simulink model "CLLCTestHarnessPlant"  (R2026a)
settings: Solver=ode23t  StopTime=5e-3  FixedStep=1e-4  MaxStep=1e-6  AbsTol=1e-3
PreLoadFcn:
  | CLLCConverterDefaultInputParameters;
undefined symbols (not defined in the file or in its folder): CLLCCompensator, CLLCController, CLLCDesign, DiscIntNeverNeededParam
libraries: fl_lib x46, nesl_utility x45, ee_lib x35
(part 2 of 4)

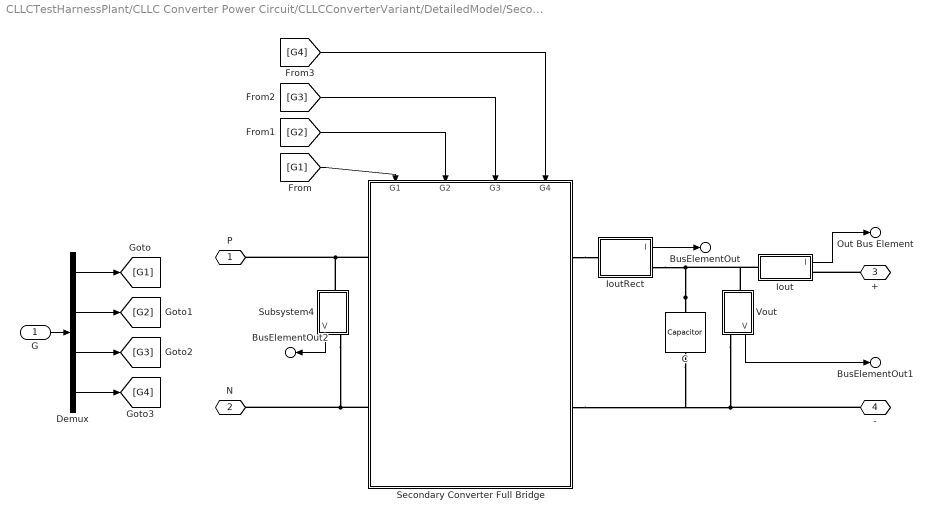
== system CLLCTestHarnessPlant/CLLC Converter Power Circuit/CLLCConverterVariant/DetailedModel/Secondary Converter ==
  G : Inport
  C : fl_lib/Electrical/Electrical Elements/Capacitor  c=Co F  r=Rco Ohm  g=0 1/Ohm  i_specify=off  i_priority=None  i=0 A  i_nominal_specify=off  i_nominal_value=1  i_nominal_unit=A  v_specify=off  v_priority=None  v=450 V  v_nominal_specify=off  v_nominal_value=1  v_nominal_unit=V  vc_specify=on  vc_priority=High  vc=Vco V  vc_nominal_specify=off  vc_nominal_value=1  vc_nominal_unit=V
  Demux : Demux
  Iout : Subsystem
      mask Display: disp("I")
  IoutRect : Subsystem
      mask Display: disp("I")
  Secondary Converter Full Bridge : Subsystem  Variant=on  VariantControlMode=label  LabelModeActiveChoice=IdealSwitch
      settings: PortSchema="{\"entries\":[{\"content\":{\"sides\":[{\"content\":{\"connectorIds\":[\"LConn1\",\"LConn2\"]},\"type\":\"ConnectorPlacement.EquallySpacedRectSide\",\"uuid\":\"27c41940-d662-4779-afdd-48b642f77411\"},{\"content\":{\"connectorIds\":[\"RConn1\",\"RConn2\"],\"side\":\"RIGHT\"},\"type\":\"ConnectorPlacement.EquallySpacedRectSide\",\"uuid\":\"b0072b01-add1-4b0f-b94e-e1b6c9886b0e\"},{\"content\":{\"connectorIds\":[\"In1\",\"In2\",\"In3\",\"In4\"],\"side\":\"TOP\"},\"type\":\"ConnectorPlacement.EquallySpacedRectSide\",\"uuid\":\"c43bed80-422d-49db-9596-8b38d5c3e411\"},{\"content\":{\"side\":\"BOTTOM\"},\"type\":\"ConnectorPlacement.EquallySpacedRectSide\",\"uuid\":\"01f06046-f57e-45b0-bca5-368a5a543f97\"}]},\"type\":\"ConnectorPlacement.EquallySpacedConnector\",\"uuid\":\"2fcb5370-6bd7-4702-bf87-ebedbb7e376c\"}],\"packageUris\":[\"http://schema.mathworks.com/mf0/Connector/R2020b\"],\"version\":\"1.0\"}"
  Subsystem4 : Subsystem
      settings: PortSchema="{\"entries\":[{\"content\":{\"sides\":[{\"content\":{\"connectorIds\":[\"LConn1\"]},\"type\":\"ConnectorPlacement.EquallySpacedRectSide\",\"uuid\":\"e749c2ff-fd60-426f-a769-b61a7dfe80d2\"},{\"content\":{\"connectorIds\":[\"RConn1\",\"Out1\"],\"side\":\"RIGHT\"},\"type\":\"ConnectorPlacement.EquallySpacedRectSide\",\"uuid\":\"f3bb02bd-f8d2-4326-b68c-6f969fa4ac22\"},{\"content\":{\"side\":\"TOP\"},\"type\":\"ConnectorPlacement.EquallySpacedRectSide\",\"uuid\":\"9ab7a0d1-20d8-49e4-8eb3-54d34434204c\"}]},\"type\":\"ConnectorPlacement.EquallySpacedConnector\",\"uuid\":\"19e2a6d5-13f4-47de-bb59-b826817cba83\"}],\"packageUris\":[\"http://schema.mathworks.com/mf0/Connector/R2020b\"],\"version\":\"1.0\"}"
      mask Display: disp("V")
  Vout : Subsystem
      settings: PortSchema="{\"entries\":[{\"content\":{\"sides\":[{\"content\":{\"connectorIds\":[\"LConn1\"]},\"type\":\"ConnectorPlacement.EquallySpacedRectSide\",\"uuid\":\"e749c2ff-fd60-426f-a769-b61a7dfe80d2\"},{\"content\":{\"connectorIds\":[\"RConn1\",\"Out1\"],\"side\":\"RIGHT\"},\"type\":\"ConnectorPlacement.EquallySpacedRectSide\",\"uuid\":\"f3bb02bd-f8d2-4326-b68c-6f969fa4ac22\"},{\"content\":{\"side\":\"TOP\"},\"type\":\"ConnectorPlacement.EquallySpacedRectSide\",\"uuid\":\"9ab7a0d1-20d8-49e4-8eb3-54d34434204c\"}]},\"type\":\"ConnectorPlacement.EquallySpacedConnector\",\"uuid\":\"19e2a6d5-13f4-47de-bb59-b826817cba83\"}],\"packageUris\":[\"http://schema.mathworks.com/mf0/Connector/R2020b\"],\"version\":\"1.0\"}"
      mask Display: disp("V")
  P : PMIOPort  Side=Left
  N : PMIOPort  Port=2  Side=Left
  + : PMIOPort  Port=3  Side=Right
  - : PMIOPort  Port=4  Side=Right
  Out Bus Element : Outport  PortName=meas  Element=Iout [A]
  BusElementOut : Outport  PortName=meas  Element=IL [A]
  BusElementOut1 : Outport  PortName=meas  Element=Vout [V]
  BusElementOut2 : Outport  PortName=meas  Element=Vac [V]
  wires:
  [G4] -> Secondary Converter Full Bridge/4(G4)
  [G1] -> Secondary Converter Full Bridge/1(G1)
  [G3] -> Secondary Converter Full Bridge/3(G3)
  [G2] -> Secondary Converter Full Bridge/2(G2)
  Demux/3 -> [G3]
  Demux/4 -> [G4]
  G/1 -> Demux/1
  Demux/1 -> [G1]
  Demux/2 -> [G2]
  Subsystem4/1(V) -> BusElementOut2/1
  Vout/1(V) -> BusElementOut1/1
  IoutRect/1(I) -> BusElementOut/1
  Iout/1(I) -> Out Bus Element/1
  connections:
  +/RConn1 -- Iout/RConn1
  C/LConn1 -- Vout/LConn1 -- Iout/LConn1 -- IoutRect/RConn1
  -/RConn1 -- Secondary Converter Full Bridge/RConn2 -- C/RConn1 -- Vout/RConn1
  Subsystem4/LConn1 -- Secondary Converter Full Bridge/LConn1 -- P/RConn1
  Subsystem4/RConn1 -- Secondary Converter Full Bridge/LConn2 -- N/RConn1
  Secondary Converter Full Bridge/RConn1 -- IoutRect/LConn1

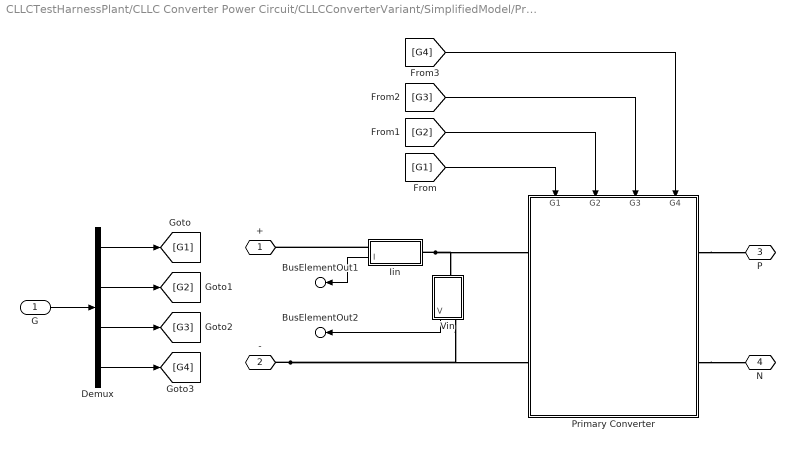
== system CLLCTestHarnessPlant/CLLC Converter Power Circuit/CLLCConverterVariant/SimplifiedModel/Primary Converter ==
  G : Inport
  Demux : Demux
  Iin : Subsystem
      settings: PortSchema="{\"entries\":[{\"content\":{\"sides\":[{\"content\":{\"connectorIds\":[\"LConn1\",\"Out1\"]},\"type\":\"ConnectorPlacement.EquallySpacedRectSide\",\"uuid\":\"e749c2ff-fd60-426f-a769-b61a7dfe80d2\"},{\"content\":{\"connectorIds\":[\"RConn1\"],\"side\":\"RIGHT\"},\"type\":\"ConnectorPlacement.EquallySpacedRectSide\",\"uuid\":\"f3bb02bd-f8d2-4326-b68c-6f969fa4ac22\"},{\"content\":{\"side\":\"TOP\"},\"type\":\"ConnectorPlacement.EquallySpacedRectSide\",\"uuid\":\"9ab7a0d1-20d8-49e4-8eb3-54d34434204c\"}]},\"type\":\"ConnectorPlacement.EquallySpacedConnector\",\"uuid\":\"19e2a6d5-13f4-47de-bb59-b826817cba83\"}],\"packageUris\":[\"http://schema.mathworks.com/mf0/Connector/R2020b\"],\"version\":\"1.0\"}"
      mask Display: disp("I")
  Primary Converter : Subsystem  VariantControl=IdealSwitch
      settings: PortSchema="{\"entries\":[{\"content\":{\"sides\":[{\"content\":{\"connectorIds\":[\"LConn1\",\"LConn2\"]},\"type\":\"ConnectorPlacement.EquallySpacedRectSide\",\"uuid\":\"27c41940-d662-4779-afdd-48b642f77411\"},{\"content\":{\"connectorIds\":[\"RConn1\",\"RConn2\"],\"side\":\"RIGHT\"},\"type\":\"ConnectorPlacement.EquallySpacedRectSide\",\"uuid\":\"b0072b01-add1-4b0f-b94e-e1b6c9886b0e\"},{\"content\":{\"connectorIds\":[\"In1\",\"In2\",\"In3\",\"In4\"],\"side\":\"TOP\"},\"type\":\"ConnectorPlacement.EquallySpacedRectSide\",\"uuid\":\"c43bed80-422d-49db-9596-8b38d5c3e411\"},{\"content\":{\"side\":\"BOTTOM\"},\"type\":\"ConnectorPlacement.EquallySpacedRectSide\",\"uuid\":\"01f06046-f57e-45b0-bca5-368a5a543f97\"}]},\"type\":\"ConnectorPlacement.EquallySpacedConnector\",\"uuid\":\"2fcb5370-6bd7-4702-bf87-ebedbb7e376c\"}],\"packageUris\":[\"http://schema.mathworks.com/mf0/Connector/R2020b\"],\"version\":\"1.0\"}"
  Vin : Subsystem
      mask Display: disp("V")
  + : PMIOPort  Side=Left
  - : PMIOPort  Port=2  Side=Left
  P : PMIOPort  Port=3  Side=Right
  N : PMIOPort  Port=4  Side=Right
  BusElementOut2 : Outport  PortName=meas  Element=Vin [V]
  BusElementOut1 : Outport  PortName=meas  Element=Iin [A]
  wires:
  [G4] -> Primary Converter/4(G4)
  [G3] -> Primary Converter/3(G3)
  [G2] -> Primary Converter/2(G2)
  [G1] -> Primary Converter/1(G1)
  G/1 -> Demux/1
  Demux/1 -> [G1]
  Demux/2 -> [G2]
  Demux/3 -> [G3]
  Demux/4 -> [G4]
  Vin/1(V) -> BusElementOut2/1
  Iin/1(I) -> BusElementOut1/1
  connections:
  Primary Converter/RConn2 -- N/RConn1
  Primary Converter/RConn1 -- P/RConn1
  -/RConn1 -- Primary Converter/LConn2 -- Vin/RConn1
  Iin/RConn1 -- Primary Converter/LConn1 -- Vin/LConn1
  Iin/LConn1 -- +/RConn1

== system CLLCTestHarnessPlant/CLLC Converter Power Circuit/CLLCConverterVariant/SimplifiedModel/Resonant Tank ==
  C1 : fl_lib/Electrical/Electrical Elements/Capacitor  c=C1 F  r=Rcr1 Ohm  g=0 1/Ohm  i_specify=off  i_priority=None  i=0 A  i_nominal_specify=off  i_nominal_value=1  i_nominal_unit=A  v_specify=off  v_priority=None  v=0 V  v_nominal_specify=off  v_nominal_value=1  v_nominal_unit=V  vc_specify=off  vc_priority=None  vc=0 V  vc_nominal_specify=off  vc_nominal_value=1  vc_nominal_unit=V
  C2 : fl_lib/Electrical/Electrical Elements/Capacitor  c=C2 F  r=Rcr2 Ohm  g=0 1/Ohm  i_specify=off  i_priority=None  i=0 A  i_nominal_specify=off  i_nominal_value=1  i_nominal_unit=A  v_specify=off  v_priority=None  v=0 V  v_nominal_specify=off  v_nominal_value=1  v_nominal_unit=V  vc_specify=off  vc_priority=None  vc=0 V  vc_nominal_specify=off  vc_nominal_value=1  vc_nominal_unit=V
  Ip : Subsystem
      settings: PortSchema="{\"entries\":[{\"content\":{\"sides\":[{\"content\":{\"connectorIds\":[\"Out1\",\"LConn1\"]},\"type\":\"ConnectorPlacement.EquallySpacedRectSide\",\"uuid\":\"e749c2ff-fd60-426f-a769-b61a7dfe80d2\"},{\"content\":{\"connectorIds\":[\"RConn1\"],\"side\":\"RIGHT\"},\"type\":\"ConnectorPlacement.EquallySpacedRectSide\",\"uuid\":\"f3bb02bd-f8d2-4326-b68c-6f969fa4ac22\"},{\"content\":{\"side\":\"TOP\"},\"type\":\"ConnectorPlacement.EquallySpacedRectSide\",\"uuid\":\"9ab7a0d1-20d8-49e4-8eb3-54d34434204c\"}]},\"type\":\"ConnectorPlacement.EquallySpacedConnector\",\"uuid\":\"19e2a6d5-13f4-47de-bb59-b826817cba83\"}],\"packageUris\":[\"http://schema.mathworks.com/mf0/Connector/R2020b\"],\"version\":\"1.0\"}"
      mask Display: disp("I")
  Is : Subsystem
      settings: PortSchema="{\"entries\":[{\"content\":{\"sides\":[{\"content\":{\"connectorIds\":[\"LConn1\"]},\"type\":\"ConnectorPlacement.EquallySpacedRectSide\",\"uuid\":\"e749c2ff-fd60-426f-a769-b61a7dfe80d2\"},{\"content\":{\"connectorIds\":[\"RConn1\",\"Out1\"],\"side\":\"RIGHT\"},\"type\":\"ConnectorPlacement.EquallySpacedRectSide\",\"uuid\":\"f3bb02bd-f8d2-4326-b68c-6f969fa4ac22\"},{\"content\":{\"side\":\"TOP\"},\"type\":\"ConnectorPlacement.EquallySpacedRectSide\",\"uuid\":\"9ab7a0d1-20d8-49e4-8eb3-54d34434204c\"}]},\"type\":\"ConnectorPlacement.EquallySpacedConnector\",\"uuid\":\"19e2a6d5-13f4-47de-bb59-b826817cba83\"}],\"packageUris\":[\"http://schema.mathworks.com/mf0/Connector/R2020b\"],\"version\":\"1.0\"}"
      mask Display: disp("I")
  Resonant Transformer : ee_lib/Passive/Transformers/Mutual Inductor  L1=Lm+Llk1 H  L2=Lm/(N1/N2)^2+Llk2 H  k=Lm/sqrt((Lm+Llk1)*(Lm+(N1/N2)^2*Llk2))  L_tol=20  enable_L1_tol=ee.enum.toleranceApplication.none  L1_tol_distribution=ee.enum.toleranceDistribution.uniform  L1_nSigma=4  enable_L2_tol=ee.enum.toleranceApplication.none  L2_tol_distribution=ee.enum.toleranceDistribution.uniform  L2_nSigma=4  r=[R1, R2] Ohm  g=[1e-09, 1e-09] 1/Ohm  enable_operating_limits=ee.enum.enable.no  operating_limit_action=ee.enum.passive.reportOpLim.warn  max_working_current=1 A  power_rating=1 W  iL1_specify=off  iL1_priority=High  iL1=0 A  iL1_nominal_specify=off  iL1_nominal_value=1  iL1_nominal_unit=A  iL2_specify=off  iL2_priority=High  iL2=0 A  iL2_nominal_specify=off  iL2_nominal_value=1  iL2_nominal_unit=A
  Vp : Subsystem
      mask Display: disp("V")
  Vs : Subsystem
      mask Display: disp("V")
  P1 : PMIOPort  Side=Left
  N1 : PMIOPort  Port=2  Side=Left
  P2 : PMIOPort  Port=3  Side=Right
  N2 : PMIOPort  Port=4  Side=Right
  Out Bus Element1 : Outport  PortName=meas  Element=Ip [A]
  Out Bus Element2 : Outport  PortName=meas  Element=Vp [V]
  Out Bus Element3 : Outport  PortName=meas  Element=Is [A]
  Out Bus Element4 : Outport  PortName=meas  Element=Vs [A]
  wires:
  Vs/1(V) -> Out Bus Element4/1
  Ip/1(I) -> Out Bus Element1/1
  Vp/1(V) -> Out Bus Element2/1
  Is/1(I) -> Out Bus Element3/1
  connections:
  Ip/LConn1 -- Vp/LConn1 -- P1/RConn1
  P2/RConn1 -- Is/RConn1 -- Vs/LConn1
  N2/RConn1 -- Resonant Transformer/RConn2 -- Vs/RConn1
  Resonant Transformer/LConn2 -- N1/RConn1 -- Vp/RConn1
  Ip/RConn1 -- C1/LConn1
  Resonant Transformer/LConn1 -- C1/RConn1
  Resonant Transformer/RConn1 -- C2/LConn1
  C2/RConn1 -- Is/LConn1

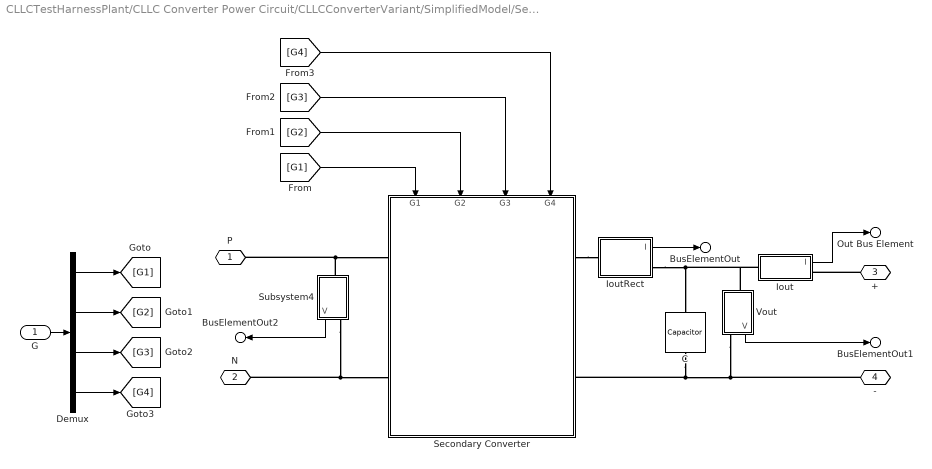
== system CLLCTestHarnessPlant/CLLC Converter Power Circuit/CLLCConverterVariant/SimplifiedModel/Secondary Converter ==
  G : Inport
  C : fl_lib/Electrical/Electrical Elements/Capacitor  c=Co F  r=Rco Ohm  g=0 1/Ohm  i_specify=off  i_priority=None  i=0 A  i_nominal_specify=off  i_nominal_value=1  i_nominal_unit=A  v_specify=off  v_priority=None  v=450 V  v_nominal_specify=off  v_nominal_value=1  v_nominal_unit=V  vc_specify=on  vc_priority=High  vc=Vco V  vc_nominal_specify=off  vc_nominal_value=1  vc_nominal_unit=V
  Demux : Demux
  Iout : Subsystem
      mask Display: disp("I")
  IoutRect : Subsystem
      mask Display: disp("I")
  Secondary Converter : Subsystem  VariantControl=IdealSwitch
      settings: PortSchema="{\"entries\":[{\"content\":{\"sides\":[{\"content\":{\"connectorIds\":[\"LConn1\",\"LConn2\"]},\"type\":\"ConnectorPlacement.EquallySpacedRectSide\",\"uuid\":\"27c41940-d662-4779-afdd-48b642f77411\"},{\"content\":{\"connectorIds\":[\"RConn1\",\"RConn2\"],\"side\":\"RIGHT\"},\"type\":\"ConnectorPlacement.EquallySpacedRectSide\",\"uuid\":\"b0072b01-add1-4b0f-b94e-e1b6c9886b0e\"},{\"content\":{\"connectorIds\":[\"In1\",\"In2\",\"In3\",\"In4\"],\"side\":\"TOP\"},\"type\":\"ConnectorPlacement.EquallySpacedRectSide\",\"uuid\":\"c43bed80-422d-49db-9596-8b38d5c3e411\"},{\"content\":{\"side\":\"BOTTOM\"},\"type\":\"ConnectorPlacement.EquallySpacedRectSide\",\"uuid\":\"01f06046-f57e-45b0-bca5-368a5a543f97\"}]},\"type\":\"ConnectorPlacement.EquallySpacedConnector\",\"uuid\":\"2fcb5370-6bd7-4702-bf87-ebedbb7e376c\"}],\"packageUris\":[\"http://schema.mathworks.com/mf0/Connector/R2020b\"],\"version\":\"1.0\"}"
  Subsystem4 : Subsystem
      settings: PortSchema="{\"entries\":[{\"content\":{\"sides\":[{\"content\":{\"connectorIds\":[\"LConn1\"]},\"type\":\"ConnectorPlacement.EquallySpacedRectSide\",\"uuid\":\"e749c2ff-fd60-426f-a769-b61a7dfe80d2\"},{\"content\":{\"connectorIds\":[\"RConn1\",\"Out1\"],\"side\":\"RIGHT\"},\"type\":\"ConnectorPlacement.EquallySpacedRectSide\",\"uuid\":\"f3bb02bd-f8d2-4326-b68c-6f969fa4ac22\"},{\"content\":{\"side\":\"TOP\"},\"type\":\"ConnectorPlacement.EquallySpacedRectSide\",\"uuid\":\"9ab7a0d1-20d8-49e4-8eb3-54d34434204c\"}]},\"type\":\"ConnectorPlacement.EquallySpacedConnector\",\"uuid\":\"19e2a6d5-13f4-47de-bb59-b826817cba83\"}],\"packageUris\":[\"http://schema.mathworks.com/mf0/Connector/R2020b\"],\"version\":\"1.0\"}"
      mask Display: disp("V")
  Vout : Subsystem
      settings: PortSchema="{\"entries\":[{\"content\":{\"sides\":[{\"content\":{\"connectorIds\":[\"LConn1\"]},\"type\":\"ConnectorPlacement.EquallySpacedRectSide\",\"uuid\":\"e749c2ff-fd60-426f-a769-b61a7dfe80d2\"},{\"content\":{\"connectorIds\":[\"RConn1\",\"Out1\"],\"side\":\"RIGHT\"},\"type\":\"ConnectorPlacement.EquallySpacedRectSide\",\"uuid\":\"f3bb02bd-f8d2-4326-b68c-6f969fa4ac22\"},{\"content\":{\"side\":\"TOP\"},\"type\":\"ConnectorPlacement.EquallySpacedRectSide\",\"uuid\":\"9ab7a0d1-20d8-49e4-8eb3-54d34434204c\"}]},\"type\":\"ConnectorPlacement.EquallySpacedConnector\",\"uuid\":\"19e2a6d5-13f4-47de-bb59-b826817cba83\"}],\"packageUris\":[\"http://schema.mathworks.com/mf0/Connector/R2020b\"],\"version\":\"1.0\"}"
      mask Display: disp("V")
  P : PMIOPort  Side=Left
  N : PMIOPort  Port=2  Side=Left
  + : PMIOPort  Port=3  Side=Right
  - : PMIOPort  Port=4  Side=Right
  Out Bus Element : Outport  PortName=meas  Element=Iout [A]
  BusElementOut : Outport  PortName=meas  Element=IL [A]
  BusElementOut1 : Outport  PortName=meas  Element=Vout [V]
  BusElementOut2 : Outport  PortName=meas  Element=Vac [V]
  wires:
  Iout/1(I) -> Out Bus Element/1
  IoutRect/1(I) -> BusElementOut/1
  Vout/1(V) -> BusElementOut1/1
  Subsystem4/1(V) -> BusElementOut2/1
  Demux/2 -> [G2]
  Demux/1 -> [G1]
  G/1 -> Demux/1
  Demux/4 -> [G4]
  Demux/3 -> [G3]
  [G2] -> Secondary Converter/2(G2)
  [G3] -> Secondary Converter/3(G3)
  [G1] -> Secondary Converter/1(G1)
  [G4] -> Secondary Converter/4(G4)
  connections:
  Secondary Converter/RConn1 -- IoutRect/LConn1
  Subsystem4/RConn1 -- N/RConn1 -- Secondary Converter/LConn2
  Subsystem4/LConn1 -- P/RConn1 -- Secondary Converter/LConn1
  C/RConn1 -- -/RConn1 -- Vout/RConn1 -- Secondary Converter/RConn2
  IoutRect/RConn1 -- Iout/LConn1 -- Vout/LConn1 -- C/LConn1
  +/RConn1 -- Iout/RConn1

== system CLLCTestHarnessPlant/CLLC PWM Generator/Primary Gate Signal/Ramp Mode/FixedStep ==
  Tsw : Inport
  Initial Ramp Value : InitialCondition  Value=0
  Overshoot Residual : Sum  Inputs=-+
  Period Reached : RelationalOperator  Operator=>  ZeroCross=off
  Time Ramp : DiscreteIntegrator  ExternalReset=rising  InitialConditionSource=external  SampleTime=Ts  ShowStatePort=on  ICPrevOutput=DiscIntNeverNeededParam  ICPrevScaledInput=DiscIntNeverNeededParam
  Unit Rate : Constant
  S : Outport
  wires:
  Initial Ramp Value/1 -> Time Ramp/3
  Overshoot Residual/1 -> Initial Ramp Value/1
  Time Ramp/State -> Overshoot Residual/2, Period Reached/1
  Tsw/1 -> Period Reached/2, Overshoot Residual/1
  Time Ramp/1 -> S/1
  Period Reached/1 -> Time Ramp/2
  Unit Rate/1 -> Time Ramp/1

== system CLLCTestHarnessPlant/CLLC PWM Generator/Primary Gate Signal/Ramp Mode/VariableStep ==
  Tsw : Inport
  Initial Ramp Value : InitialCondition  Value=0
  Overshoot Residual : Sum  Inputs=-+
  Period Reached : RelationalOperator  Operator=>
  Time Ramp : Integrator  ExternalReset=rising  InitialConditionSource=external  ShowStatePort=on
  Unit Rate : Constant
  S : Outport
  wires:
  Initial Ramp Value/1 -> Time Ramp/3
  Overshoot Residual/1 -> Initial Ramp Value/1
  Time Ramp/State -> Overshoot Residual/2, Period Reached/1
  Tsw/1 -> Period Reached/2, Overshoot Residual/1
  Time Ramp/1 -> S/1
  Period Reached/1 -> Time Ramp/2
  Unit Rate/1 -> Time Ramp/1

== system CLLCTestHarnessPlant/CLLC PWM Generator/Synchronous Rectifier/Region Select/Above Resonance ==
  primaryGates : Inport
  permit : Inport  Port=2
  Action Port : ActionPort  ActionPortLabel=elseif(u1 >= fpuSrUpper)
  Unused Primary Gates : Terminator
  Gs : Outport  InitialOutput=0
  wires:
  permit/1 -> Gs/1
  primaryGates/1 -> Unused Primary Gates/1

== system CLLCTestHarnessPlant/CLLC PWM Generator/Synchronous Rectifier/Region Select/Below Resonance ==
  primaryGates : Inport
  permit : Inport  Port=2
  Action Port : ActionPort  ActionPortLabel=if(u1 <= fpuSrLower)
  Rectifier Permit : Logic
  Gs : Outport  InitialOutput=0
  wires:
  Rectifier Permit/1 -> Gs/1
  permit/1 -> Rectifier Permit/2
  primaryGates/1 -> Rectifier Permit/1

== system CLLCTestHarnessPlant/CLLC PWM Generator/Synchronous Rectifier/Region Select/Within Band ==
  primaryGates : Inport
  permit : Inport  Port=2
  Action Port : ActionPort  ActionPortLabel=else
  Unused Rectifier Permit : Terminator
  Gs : Outport  InitialOutput=0
  wires:
  primaryGates/1 -> Gs/1
  permit/1 -> Unused Rectifier Permit/1

== system CLLCTestHarnessPlant/CLLC PWM Generator/Synchronous Rectifier/Turn On Delay/Rectifier Ramp Mode ==
  rate : Inport
  FixedStep : Subsystem  VariantControl=FixedStep
  VariableStep : Subsystem  VariantControl=VariableStep
  S : Outport

== system CLLCTestHarnessPlant/CLLC Converter Power Circuit/CLLCConverterVariant/DetailedModel/Primary Converter/Iin ==
  Current Sensor : fl_lib/Electrical/Electrical Sensors/Current Sensor
  PS-Simulink Converter : nesl_utility/PS-Simulink Converter  PhysicalDomain=network_engine_domain  SubClassName=ps_output  LeftPortType=input  RightPortType=output  PseudoPeriodic=off  Frequencies=[]  VectorFormat=inherit  Unit=inherit  AffineConversion=off
  + : PMIOPort  Side=Left
  - : PMIOPort  Port=2  Side=Right
  I : Outport
  wires:
  PS-Simulink Converter/1 -> I/1
  connections:
  Current Sensor/RConn2 -- -/RConn1
  +/RConn1 -- Current Sensor/LConn1
  Current Sensor/RConn1 -- PS-Simulink Converter/LConn1

== system CLLCTestHarnessPlant/CLLC Converter Power Circuit/CLLCConverterVariant/DetailedModel/Primary Converter/Primary Converter Full Bridge ==
  G1 : Inport
  G2 : Inport  Port=2
  G3 : Inport  Port=3
  G4 : Inport  Port=4
  Ideal MOSFET with Thermal : Subsystem  VariantControl=IdealMOSFETwithThermal
      settings: PortSchema="{\"entries\":[{\"content\":{\"sides\":[{\"content\":{\"connectorIds\":[\"LConn1\",\"LConn2\"]},\"type\":\"ConnectorPlacement.EquallySpacedRectSide\",\"uuid\":\"27c41940-d662-4779-afdd-48b642f77411\"},{\"content\":{\"connectorIds\":[\"RConn1\",\"RConn2\"],\"side\":\"RIGHT\"},\"type\":\"ConnectorPlacement.EquallySpacedRectSide\",\"uuid\":\"b0072b01-add1-4b0f-b94e-e1b6c9886b0e\"},{\"content\":{\"connectorIds\":[\"In1\",\"In2\",\"In3\",\"In4\"],\"side\":\"TOP\"},\"type\":\"ConnectorPlacement.EquallySpacedRectSide\",\"uuid\":\"c43bed80-422d-49db-9596-8b38d5c3e411\"},{\"content\":{\"side\":\"BOTTOM\"},\"type\":\"ConnectorPlacement.EquallySpacedRectSide\",\"uuid\":\"01f06046-f57e-45b0-bca5-368a5a543f97\"}]},\"type\":\"ConnectorPlacement.EquallySpacedConnector\",\"uuid\":\"2fcb5370-6bd7-4702-bf87-ebedbb7e376c\"}],\"packageUris\":[\"http://schema.mathworks.com/mf0/Connector/R2020b\"],\"version\":\"1.0\"}"
  Ideal Switch : Subsystem  VariantControl=IdealSwitch
      settings: PortSchema="{\"entries\":[{\"content\":{\"sides\":[{\"content\":{\"connectorIds\":[\"LConn1\",\"LConn2\"]},\"type\":\"ConnectorPlacement.EquallySpacedRectSide\",\"uuid\":\"27c41940-d662-4779-afdd-48b642f77411\"},{\"content\":{\"connectorIds\":[\"RConn1\",\"RConn2\"],\"side\":\"RIGHT\"},\"type\":\"ConnectorPlacement.EquallySpacedRectSide\",\"uuid\":\"b0072b01-add1-4b0f-b94e-e1b6c9886b0e\"},{\"content\":{\"connectorIds\":[\"In1\",\"In2\",\"In3\",\"In4\"],\"side\":\"TOP\"},\"type\":\"ConnectorPlacement.EquallySpacedRectSide\",\"uuid\":\"c43bed80-422d-49db-9596-8b38d5c3e411\"},{\"content\":{\"side\":\"BOTTOM\"},\"type\":\"ConnectorPlacement.EquallySpacedRectSide\",\"uuid\":\"01f06046-f57e-45b0-bca5-368a5a543f97\"}]},\"type\":\"ConnectorPlacement.EquallySpacedConnector\",\"uuid\":\"2fcb5370-6bd7-4702-bf87-ebedbb7e376c\"}],\"packageUris\":[\"http://schema.mathworks.com/mf0/Connector/R2020b\"],\"version\":\"1.0\"}"
  P1 : PMIOPort  Side=Left
  N1 : PMIOPort  Port=2  Side=Left
  P2 : PMIOPort  Port=3  Side=Right
  N2 : PMIOPort  Port=4  Side=Right

== system CLLCTestHarnessPlant/CLLC Converter Power Circuit/CLLCConverterVariant/DetailedModel/Primary Converter/Vin ==
  PS-Simulink Converter : nesl_utility/PS-Simulink Converter  PhysicalDomain=network_engine_domain  SubClassName=ps_output  LeftPortType=input  RightPortType=output  PseudoPeriodic=off  Frequencies=[]  VectorFormat=inherit  Unit=inherit  AffineConversion=off
  Voltage Sensor : fl_lib/Electrical/Electrical Sensors/Voltage Sensor
  + : PMIOPort  Side=Left
  - : PMIOPort  Port=2  Side=Right
  V : Outport
  wires:
  PS-Simulink Converter/1 -> V/1
  connections:
  Voltage Sensor/RConn2 -- -/RConn1
  Voltage Sensor/LConn1 -- +/RConn1
  PS-Simulink Converter/LConn1 -- Voltage Sensor/RConn1

== system CLLCTestHarnessPlant/CLLC Converter Power Circuit/CLLCConverterVariant/DetailedModel/Resonant Tank/Ip ==
  Current Sensor : fl_lib/Electrical/Electrical Sensors/Current Sensor
  PS-Simulink Converter : nesl_utility/PS-Simulink Converter  PhysicalDomain=network_engine_domain  SubClassName=ps_output  LeftPortType=input  RightPortType=output  PseudoPeriodic=off  Frequencies=[]  VectorFormat=inherit  Unit=inherit  AffineConversion=off
  + : PMIOPort  Side=Left
  - : PMIOPort  Port=2  Side=Right
  I : Outport
  wires:
  PS-Simulink Converter/1 -> I/1
  connections:
  Current Sensor/RConn2 -- -/RConn1
  +/RConn1 -- Current Sensor/LConn1
  Current Sensor/RConn1 -- PS-Simulink Converter/LConn1

== system CLLCTestHarnessPlant/CLLC Converter Power Circuit/CLLCConverterVariant/DetailedModel/Resonant Tank/Is ==
  Current Sensor : fl_lib/Electrical/Electrical Sensors/Current Sensor
  PS-Simulink Converter : nesl_utility/PS-Simulink Converter  PhysicalDomain=network_engine_domain  SubClassName=ps_output  LeftPortType=input  RightPortType=output  PseudoPeriodic=off  Frequencies=[]  VectorFormat=inherit  Unit=inherit  AffineConversion=off
  + : PMIOPort  Side=Left
  - : PMIOPort  Port=2  Side=Right
  I : Outport
  wires:
  PS-Simulink Converter/1 -> I/1
  connections:
  Current Sensor/RConn2 -- -/RConn1
  +/RConn1 -- Current Sensor/LConn1
  Current Sensor/RConn1 -- PS-Simulink Converter/LConn1

== system CLLCTestHarnessPlant/CLLC Converter Power Circuit/CLLCConverterVariant/DetailedModel/Resonant Tank/Vp ==
  PS-Simulink Converter : nesl_utility/PS-Simulink Converter  PhysicalDomain=network_engine_domain  SubClassName=ps_output  LeftPortType=input  RightPortType=output  PseudoPeriodic=off  Frequencies=[]  VectorFormat=inherit  Unit=inherit  AffineConversion=off
  Voltage Sensor : fl_lib/Electrical/Electrical Sensors/Voltage Sensor
  + : PMIOPort  Side=Left
  - : PMIOPort  Port=2  Side=Right
  V : Outport
  wires:
  PS-Simulink Converter/1 -> V/1
  connections:
  Voltage Sensor/RConn2 -- -/RConn1
  Voltage Sensor/LConn1 -- +/RConn1
  PS-Simulink Converter/LConn1 -- Voltage Sensor/RConn1

== system CLLCTestHarnessPlant/CLLC Converter Power Circuit/CLLCConverterVariant/DetailedModel/Resonant Tank/Vs ==
  PS-Simulink Converter : nesl_utility/PS-Simulink Converter  PhysicalDomain=network_engine_domain  SubClassName=ps_output  LeftPortType=input  RightPortType=output  PseudoPeriodic=off  Frequencies=[]  VectorFormat=inherit  Unit=inherit  AffineConversion=off
  Voltage Sensor : fl_lib/Electrical/Electrical Sensors/Voltage Sensor
  + : PMIOPort  Side=Left
  - : PMIOPort  Port=2  Side=Right
  V : Outport
  wires:
  PS-Simulink Converter/1 -> V/1
  connections:
  Voltage Sensor/RConn2 -- -/RConn1
  Voltage Sensor/LConn1 -- +/RConn1
  PS-Simulink Converter/LConn1 -- Voltage Sensor/RConn1

== system CLLCTestHarnessPlant/CLLC Converter Power Circuit/CLLCConverterVariant/DetailedModel/Secondary Converter/Iout ==
  Current Sensor : fl_lib/Electrical/Electrical Sensors/Current Sensor
  PS-Simulink Converter : nesl_utility/PS-Simulink Converter  PhysicalDomain=network_engine_domain  SubClassName=ps_output  LeftPortType=input  RightPortType=output  PseudoPeriodic=off  Frequencies=[]  VectorFormat=inherit  Unit=inherit  AffineConversion=off
  + : PMIOPort  Side=Left
  - : PMIOPort  Port=2  Side=Right
  I : Outport
  wires:
  PS-Simulink Converter/1 -> I/1
  connections:
  Current Sensor/RConn2 -- -/RConn1
  +/RConn1 -- Current Sensor/LConn1
  Current Sensor/RConn1 -- PS-Simulink Converter/LConn1

== system CLLCTestHarnessPlant/CLLC Converter Power Circuit/CLLCConverterVariant/DetailedModel/Secondary Converter/IoutRect ==
  Current Sensor : fl_lib/Electrical/Electrical Sensors/Current Sensor
  PS-Simulink Converter : nesl_utility/PS-Simulink Converter  PhysicalDomain=network_engine_domain  SubClassName=ps_output  LeftPortType=input  RightPortType=output  PseudoPeriodic=off  Frequencies=[]  VectorFormat=inherit  Unit=inherit  AffineConversion=off
  + : PMIOPort  Side=Left
  - : PMIOPort  Port=2  Side=Right
  I : Outport
  wires:
  PS-Simulink Converter/1 -> I/1
  connections:
  Current Sensor/RConn2 -- -/RConn1
  +/RConn1 -- Current Sensor/LConn1
  Current Sensor/RConn1 -- PS-Simulink Converter/LConn1

== system CLLCTestHarnessPlant/CLLC Converter Power Circuit/CLLCConverterVariant/DetailedModel/Secondary Converter/Secondary Converter Full Bridge ==
  G1 : Inport
  G2 : Inport  Port=2
  G3 : Inport  Port=3
  G4 : Inport  Port=4
  Ideal MOSFET with Thermal : Subsystem  VariantControl=IdealMOSFETwithThermal
      settings: PortSchema="{\"entries\":[{\"content\":{\"sides\":[{\"content\":{\"connectorIds\":[\"LConn1\",\"LConn2\"]},\"type\":\"ConnectorPlacement.EquallySpacedRectSide\",\"uuid\":\"27c41940-d662-4779-afdd-48b642f77411\"},{\"content\":{\"connectorIds\":[\"RConn1\",\"RConn2\"],\"side\":\"RIGHT\"},\"type\":\"ConnectorPlacement.EquallySpacedRectSide\",\"uuid\":\"b0072b01-add1-4b0f-b94e-e1b6c9886b0e\"},{\"content\":{\"connectorIds\":[\"In1\",\"In2\",\"In3\",\"In4\"],\"side\":\"TOP\"},\"type\":\"ConnectorPlacement.EquallySpacedRectSide\",\"uuid\":\"c43bed80-422d-49db-9596-8b38d5c3e411\"},{\"content\":{\"side\":\"BOTTOM\"},\"type\":\"ConnectorPlacement.EquallySpacedRectSide\",\"uuid\":\"01f06046-f57e-45b0-bca5-368a5a543f97\"}]},\"type\":\"ConnectorPlacement.EquallySpacedConnector\",\"uuid\":\"2fcb5370-6bd7-4702-bf87-ebedbb7e376c\"}],\"packageUris\":[\"http://schema.mathworks.com/mf0/Connector/R2020b\"],\"version\":\"1.0\"}"
  Ideal Switch : Subsystem  VariantControl=IdealSwitch
      settings: PortSchema="{\"entries\":[{\"content\":{\"sides\":[{\"content\":{\"connectorIds\":[\"LConn1\",\"LConn2\"]},\"type\":\"ConnectorPlacement.EquallySpacedRectSide\",\"uuid\":\"27c41940-d662-4779-afdd-48b642f77411\"},{\"content\":{\"connectorIds\":[\"RConn1\",\"RConn2\"],\"side\":\"RIGHT\"},\"type\":\"ConnectorPlacement.EquallySpacedRectSide\",\"uuid\":\"b0072b01-add1-4b0f-b94e-e1b6c9886b0e\"},{\"content\":{\"connectorIds\":[\"In1\",\"In2\",\"In3\",\"In4\"],\"side\":\"TOP\"},\"type\":\"ConnectorPlacement.EquallySpacedRectSide\",\"uuid\":\"c43bed80-422d-49db-9596-8b38d5c3e411\"},{\"content\":{\"side\":\"BOTTOM\"},\"type\":\"ConnectorPlacement.EquallySpacedRectSide\",\"uuid\":\"01f06046-f57e-45b0-bca5-368a5a543f97\"}]},\"type\":\"ConnectorPlacement.EquallySpacedConnector\",\"uuid\":\"2fcb5370-6bd7-4702-bf87-ebedbb7e376c\"}],\"packageUris\":[\"http://schema.mathworks.com/mf0/Connector/R2020b\"],\"version\":\"1.0\"}"
  P1 : PMIOPort  Side=Right
  N1 : PMIOPort  Port=2  Side=Right
  P2 : PMIOPort  Port=3  Side=Left
  N2 : PMIOPort  Port=4  Side=Left

== system CLLCTestHarnessPlant/CLLC Converter Power Circuit/CLLCConverterVariant/DetailedModel/Secondary Converter/Subsystem4 ==
  PS-Simulink Converter : nesl_utility/PS-Simulink Converter  PhysicalDomain=network_engine_domain  SubClassName=ps_output  LeftPortType=input  RightPortType=output  PseudoPeriodic=off  Frequencies=[]  VectorFormat=inherit  Unit=inherit  AffineConversion=off
  Voltage Sensor : fl_lib/Electrical/Electrical Sensors/Voltage Sensor
  + : PMIOPort  Side=Left
  - : PMIOPort  Port=2  Side=Right
  V : Outport
  wires:
  PS-Simulink Converter/1 -> V/1
  connections:
  Voltage Sensor/RConn2 -- -/RConn1
  Voltage Sensor/LConn1 -- +/RConn1
  PS-Simulink Converter/LConn1 -- Voltage Sensor/RConn1

== system CLLCTestHarnessPlant/CLLC Converter Power Circuit/CLLCConverterVariant/DetailedModel/Secondary Converter/Vout ==
  PS-Simulink Converter : nesl_utility/PS-Simulink Converter  PhysicalDomain=network_engine_domain  SubClassName=ps_output  LeftPortType=input  RightPortType=output  PseudoPeriodic=off  Frequencies=[]  VectorFormat=inherit  Unit=inherit  AffineConversion=off
  Voltage Sensor : fl_lib/Electrical/Electrical Sensors/Voltage Sensor
  + : PMIOPort  Side=Left
  - : PMIOPort  Port=2  Side=Right
  V : Outport
  wires:
  PS-Simulink Converter/1 -> V/1
  connections:
  Voltage Sensor/RConn2 -- -/RConn1
  Voltage Sensor/LConn1 -- +/RConn1
  PS-Simulink Converter/LConn1 -- Voltage Sensor/RConn1

== system CLLCTestHarnessPlant/CLLC Converter Power Circuit/CLLCConverterVariant/SimplifiedModel/Primary Converter/Iin ==
  Current Sensor : fl_lib/Electrical/Electrical Sensors/Current Sensor
  PS-Simulink Converter : nesl_utility/PS-Simulink Converter  PhysicalDomain=network_engine_domain  SubClassName=ps_output  LeftPortType=input  RightPortType=output  PseudoPeriodic=off  Frequencies=[]  VectorFormat=inherit  Unit=inherit  AffineConversion=off
  + : PMIOPort  Side=Left
  - : PMIOPort  Port=2  Side=Right
  I : Outport
  wires:
  PS-Simulink Converter/1 -> I/1
  connections:
  Current Sensor/RConn1 -- PS-Simulink Converter/LConn1
  +/RConn1 -- Current Sensor/LConn1
  Current Sensor/RConn2 -- -/RConn1

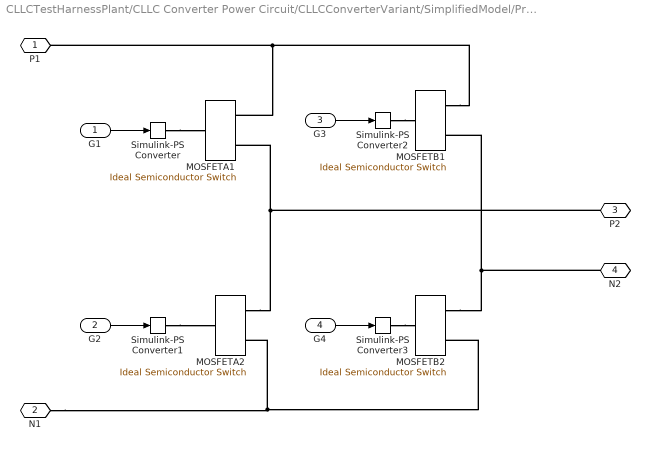
== system CLLCTestHarnessPlant/CLLC Converter Power Circuit/CLLCConverterVariant/SimplifiedModel/Primary Converter/Primary Converter ==
  G1 : Inport
  G2 : Inport  Port=2
  G3 : Inport  Port=3
  G4 : Inport  Port=4
  MOSFETA1 : ee_lib/Semiconductors & Converters/Ideal Semiconductor Switch  port_option=ee.enum.controlport.ps  Ron=PrimaryRon Ohm  Goff=PrimaryGoff 1/Ohm  Vth=PrimaryVth V  diode_param=ee.enum.semiconductors.protectionDiode.nodynamics  diode_Vf=PrimaryVbodydiodeOn V  diode_Ron=PrimaryRbodydiodeOn Ohm  diode_Goff=PrimaryGbodydiodeOff 1/Ohm  diode_C=50e-9 F  diode_iRM=-235 A  diode_iF=300 A  diode_idot=-50 A/us  diode_trr_param=ee.enum.converters.diodetrr.trr_factor  diode_trr_factor=3  diode_trr=15 us  diode_Qrr=1500 s*uA
  MOSFETA2 : ee_lib/Semiconductors & Converters/Ideal Semiconductor Switch  port_option=ee.enum.controlport.ps  Ron=PrimaryRon Ohm  Goff=PrimaryGoff 1/Ohm  Vth=PrimaryVth V  diode_param=ee.enum.semiconductors.protectionDiode.nodynamics  diode_Vf=PrimaryVbodydiodeOn V  diode_Ron=PrimaryRbodydiodeOn Ohm  diode_Goff=PrimaryGbodydiodeOff 1/Ohm  diode_C=50e-9 F  diode_iRM=-235 A  diode_iF=300 A  diode_idot=-50 A/us  diode_trr_param=ee.enum.converters.diodetrr.trr_factor  diode_trr_factor=3  diode_trr=15 us  diode_Qrr=1500 s*uA
  MOSFETB1 : ee_lib/Semiconductors & Converters/Ideal Semiconductor Switch  port_option=ee.enum.controlport.ps  Ron=PrimaryRon Ohm  Goff=PrimaryGoff 1/Ohm  Vth=PrimaryVth V  diode_param=ee.enum.semiconductors.protectionDiode.nodynamics  diode_Vf=PrimaryVbodydiodeOn V  diode_Ron=PrimaryRbodydiodeOn Ohm  diode_Goff=PrimaryGbodydiodeOff 1/Ohm  diode_C=50e-9 F  diode_iRM=-235 A  diode_iF=300 A  diode_idot=-50 A/us  diode_trr_param=ee.enum.converters.diodetrr.trr_factor  diode_trr_factor=3  diode_trr=15 us  diode_Qrr=1500 s*uA
  MOSFETB2 : ee_lib/Semiconductors & Converters/Ideal Semiconductor Switch  port_option=ee.enum.controlport.ps  Ron=PrimaryRon Ohm  Goff=PrimaryGoff 1/Ohm  Vth=PrimaryVth V  diode_param=ee.enum.semiconductors.protectionDiode.nodynamics  diode_Vf=PrimaryVbodydiodeOn V  diode_Ron=PrimaryRbodydiodeOn Ohm  diode_Goff=PrimaryGbodydiodeOff 1/Ohm  diode_C=50e-9 F  diode_iRM=-235 A  diode_iF=300 A  diode_idot=-50 A/us  diode_trr_param=ee.enum.converters.diodetrr.trr_factor  diode_trr_factor=3  diode_trr=15 us  diode_Qrr=1500 s*uA
  Simulink-PS Converter{,1..3} (4 alike) : nesl_utility/Simulink-PS Converter  PhysicalDomain=network_engine_domain  SubClassName=ps_input  LeftPortType=input  RightPortType=output  PseudoPeriodic=off  Frequencies=[]  NoiseDistribution=none  NoiseParameters=[]  Unit=1  AffineConversion=off  FilteringAndDerivatives=provide  SimscapeFilterOrder=1  InputFilterTimeConstant=0.001  UdotUserProvided=0
  P1 : PMIOPort  Side=Left
  N1 : PMIOPort  Port=2  Side=Left
  P2 : PMIOPort  Port=3  Side=Right
  N2 : PMIOPort  Port=4  Side=Right
  wires:
  G4/1 -> Simulink-PS Converter3/1
  G3/1 -> Simulink-PS Converter2/1
  G2/1 -> Simulink-PS Converter1/1
  G1/1 -> Simulink-PS Converter/1
  connections:
  Simulink-PS Converter3/RConn1 -- MOSFETB2/LConn1
  Simulink-PS Converter2/RConn1 -- MOSFETB1/LConn1
  Simulink-PS Converter1/RConn1 -- MOSFETA2/LConn1
  Simulink-PS Converter/RConn1 -- MOSFETA1/LConn1
  MOSFETA2/RConn2 -- MOSFETB2/RConn2 -- N1/RConn1
  MOSFETA1/RConn1 -- MOSFETB1/RConn1 -- P1/RConn1
  MOSFETA1/RConn2 -- MOSFETA2/RConn1 -- P2/RConn1
  MOSFETB1/RConn2 -- MOSFETB2/RConn1 -- N2/RConn1

== system CLLCTestHarnessPlant/CLLC Converter Power Circuit/CLLCConverterVariant/SimplifiedModel/Primary Converter/Vin ==
  PS-Simulink Converter : nesl_utility/PS-Simulink Converter  PhysicalDomain=network_engine_domain  SubClassName=ps_output  LeftPortType=input  RightPortType=output  PseudoPeriodic=off  Frequencies=[]  VectorFormat=inherit  Unit=inherit  AffineConversion=off
  Voltage Sensor : fl_lib/Electrical/Electrical Sensors/Voltage Sensor
  + : PMIOPort  Side=Left
  - : PMIOPort  Port=2  Side=Right
  V : Outport
  wires:
  PS-Simulink Converter/1 -> V/1
  connections:
  PS-Simulink Converter/LConn1 -- Voltage Sensor/RConn1
  Voltage Sensor/LConn1 -- +/RConn1
  Voltage Sensor/RConn2 -- -/RConn1

== system CLLCTestHarnessPlant/CLLC Converter Power Circuit/CLLCConverterVariant/SimplifiedModel/Resonant Tank/Ip ==
  Current Sensor : fl_lib/Electrical/Electrical Sensors/Current Sensor
  PS-Simulink Converter : nesl_utility/PS-Simulink Converter  PhysicalDomain=network_engine_domain  SubClassName=ps_output  LeftPortType=input  RightPortType=output  PseudoPeriodic=off  Frequencies=[]  VectorFormat=inherit  Unit=inherit  AffineConversion=off
  + : PMIOPort  Side=Left
  - : PMIOPort  Port=2  Side=Right
  I : Outport
  wires:
  PS-Simulink Converter/1 -> I/1
  connections:
  Current Sensor/RConn1 -- PS-Simulink Converter/LConn1
  +/RConn1 -- Current Sensor/LConn1
  Current Sensor/RConn2 -- -/RConn1

== system CLLCTestHarnessPlant/CLLC Converter Power Circuit/CLLCConverterVariant/SimplifiedModel/Resonant Tank/Is ==
  Current Sensor : fl_lib/Electrical/Electrical Sensors/Current Sensor
  PS-Simulink Converter : nesl_utility/PS-Simulink Converter  PhysicalDomain=network_engine_domain  SubClassName=ps_output  LeftPortType=input  RightPortType=output  PseudoPeriodic=off  Frequencies=[]  VectorFormat=inherit  Unit=inherit  AffineConversion=off
  + : PMIOPort  Side=Left
  - : PMIOPort  Port=2  Side=Right
  I : Outport
  wires:
  PS-Simulink Converter/1 -> I/1
  connections:
  Current Sensor/RConn1 -- PS-Simulink Converter/LConn1
  +/RConn1 -- Current Sensor/LConn1
  Current Sensor/RConn2 -- -/RConn1

== system CLLCTestHarnessPlant/CLLC Converter Power Circuit/CLLCConverterVariant/SimplifiedModel/Resonant Tank/Vp ==
  PS-Simulink Converter : nesl_utility/PS-Simulink Converter  PhysicalDomain=network_engine_domain  SubClassName=ps_output  LeftPortType=input  RightPortType=output  PseudoPeriodic=off  Frequencies=[]  VectorFormat=inherit  Unit=inherit  AffineConversion=off
  Voltage Sensor : fl_lib/Electrical/Electrical Sensors/Voltage Sensor
  + : PMIOPort  Side=Left
  - : PMIOPort  Port=2  Side=Right
  V : Outport
  wires:
  PS-Simulink Converter/1 -> V/1
  connections:
  PS-Simulink Converter/LConn1 -- Voltage Sensor/RConn1
  Voltage Sensor/LConn1 -- +/RConn1
  Voltage Sensor/RConn2 -- -/RConn1

== system CLLCTestHarnessPlant/CLLC Converter Power Circuit/CLLCConverterVariant/SimplifiedModel/Resonant Tank/Vs ==
  PS-Simulink Converter : nesl_utility/PS-Simulink Converter  PhysicalDomain=network_engine_domain  SubClassName=ps_output  LeftPortType=input  RightPortType=output  PseudoPeriodic=off  Frequencies=[]  VectorFormat=inherit  Unit=inherit  AffineConversion=off
  Voltage Sensor : fl_lib/Electrical/Electrical Sensors/Voltage Sensor
  + : PMIOPort  Side=Left
  - : PMIOPort  Port=2  Side=Right
  V : Outport
  wires:
  PS-Simulink Converter/1 -> V/1
  connections:
  PS-Simulink Converter/LConn1 -- Voltage Sensor/RConn1
  Voltage Sensor/LConn1 -- +/RConn1
  Voltage Sensor/RConn2 -- -/RConn1

== system CLLCTestHarnessPlant/CLLC Converter Power Circuit/CLLCConverterVariant/SimplifiedModel/Secondary Converter/Iout ==
  Current Sensor : fl_lib/Electrical/Electrical Sensors/Current Sensor
  PS-Simulink Converter : nesl_utility/PS-Simulink Converter  PhysicalDomain=network_engine_domain  SubClassName=ps_output  LeftPortType=input  RightPortType=output  PseudoPeriodic=off  Frequencies=[]  VectorFormat=inherit  Unit=inherit  AffineConversion=off
  + : PMIOPort  Side=Left
  - : PMIOPort  Port=2  Side=Right
  I : Outport
  wires:
  PS-Simulink Converter/1 -> I/1
  connections:
  Current Sensor/RConn1 -- PS-Simulink Converter/LConn1
  +/RConn1 -- Current Sensor/LConn1
  Current Sensor/RConn2 -- -/RConn1

== system CLLCTestHarnessPlant/CLLC Converter Power Circuit/CLLCConverterVariant/SimplifiedModel/Secondary Converter/IoutRect ==
  Current Sensor : fl_lib/Electrical/Electrical Sensors/Current Sensor
  PS-Simulink Converter : nesl_utility/PS-Simulink Converter  PhysicalDomain=network_engine_domain  SubClassName=ps_output  LeftPortType=input  RightPortType=output  PseudoPeriodic=off  Frequencies=[]  VectorFormat=inherit  Unit=inherit  AffineConversion=off
  + : PMIOPort  Side=Left
  - : PMIOPort  Port=2  Side=Right
  I : Outport
  wires:
  PS-Simulink Converter/1 -> I/1
  connections:
  Current Sensor/RConn1 -- PS-Simulink Converter/LConn1
  +/RConn1 -- Current Sensor/LConn1
  Current Sensor/RConn2 -- -/RConn1

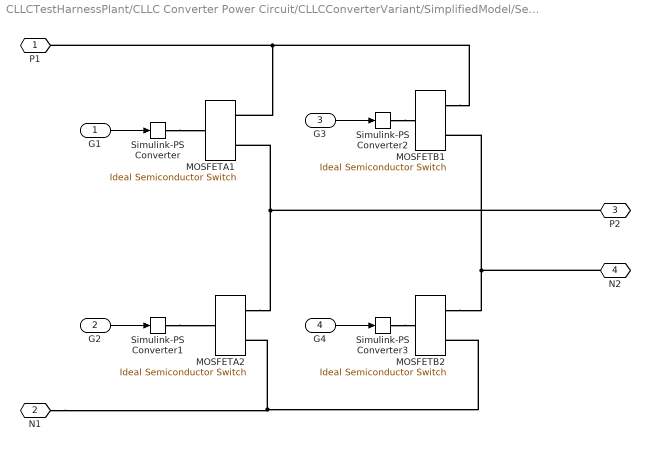
== system CLLCTestHarnessPlant/CLLC Converter Power Circuit/CLLCConverterVariant/SimplifiedModel/Secondary Converter/Secondary Converter ==
  G1 : Inport
  G2 : Inport  Port=2
  G3 : Inport  Port=3
  G4 : Inport  Port=4
  MOSFETA1 : ee_lib/Semiconductors & Converters/Ideal Semiconductor Switch  port_option=ee.enum.controlport.ps  Ron=SecondaryRon Ohm  Goff=SecondaryGoff 1/Ohm  Vth=SecondaryVth V  diode_param=ee.enum.semiconductors.protectionDiode.nodynamics  diode_Vf=SecondaryVbodydiodeOn V  diode_Ron=SecondaryRbodydiodeOn Ohm  diode_Goff=SecondaryGbodydiodeOff 1/Ohm  diode_C=50e-9 F  diode_iRM=-235 A  diode_iF=300 A  diode_idot=-50 A/us  diode_trr_param=ee.enum.converters.diodetrr.trr_factor  diode_trr_factor=3  diode_trr=15 us  diode_Qrr=1500 s*uA
  MOSFETA2 : ee_lib/Semiconductors & Converters/Ideal Semiconductor Switch  port_option=ee.enum.controlport.ps  Ron=SecondaryRon Ohm  Goff=SecondaryGoff 1/Ohm  Vth=SecondaryVth V  diode_param=ee.enum.semiconductors.protectionDiode.nodynamics  diode_Vf=SecondaryVbodydiodeOn V  diode_Ron=SecondaryRbodydiodeOn Ohm  diode_Goff=SecondaryGbodydiodeOff 1/Ohm  diode_C=50e-9 F  diode_iRM=-235 A  diode_iF=300 A  diode_idot=-50 A/us  diode_trr_param=ee.enum.converters.diodetrr.trr_factor  diode_trr_factor=3  diode_trr=15 us  diode_Qrr=1500 s*uA
  MOSFETB1 : ee_lib/Semiconductors & Converters/Ideal Semiconductor Switch  port_option=ee.enum.controlport.ps  Ron=SecondaryRon Ohm  Goff=SecondaryGoff 1/Ohm  Vth=SecondaryVth V  diode_param=ee.enum.semiconductors.protectionDiode.nodynamics  diode_Vf=SecondaryVbodydiodeOn V  diode_Ron=SecondaryRbodydiodeOn Ohm  diode_Goff=SecondaryGbodydiodeOff 1/Ohm  diode_C=50e-9 F  diode_iRM=-235 A  diode_iF=300 A  diode_idot=-50 A/us  diode_trr_param=ee.enum.converters.diodetrr.trr_factor  diode_trr_factor=3  diode_trr=15 us  diode_Qrr=1500 s*uA
  MOSFETB2 : ee_lib/Semiconductors & Converters/Ideal Semiconductor Switch  port_option=ee.enum.controlport.ps  Ron=SecondaryRon Ohm  Goff=SecondaryGoff 1/Ohm  Vth=SecondaryVth V  diode_param=ee.enum.semiconductors.protectionDiode.nodynamics  diode_Vf=SecondaryVbodydiodeOn V  diode_Ron=SecondaryRbodydiodeOn Ohm  diode_Goff=SecondaryGbodydiodeOff 1/Ohm  diode_C=50e-9 F  diode_iRM=-235 A  diode_iF=300 A  diode_idot=-50 A/us  diode_trr_param=ee.enum.converters.diodetrr.trr_factor  diode_trr_factor=3  diode_trr=15 us  diode_Qrr=1500 s*uA
  Simulink-PS Converter{,1..3} (4 alike) : nesl_utility/Simulink-PS Converter  PhysicalDomain=network_engine_domain  SubClassName=ps_input  LeftPortType=input  RightPortType=output  PseudoPeriodic=off  Frequencies=[]  NoiseDistribution=none  NoiseParameters=[]  Unit=1  AffineConversion=off  FilteringAndDerivatives=provide  SimscapeFilterOrder=1  InputFilterTimeConstant=0.001  UdotUserProvided=0
  P1 : PMIOPort  Side=Right
  N1 : PMIOPort  Port=2  Side=Right
  P2 : PMIOPort  Port=3  Side=Left
  N2 : PMIOPort  Port=4  Side=Left
  wires:
  G4/1 -> Simulink-PS Converter3/1
  G3/1 -> Simulink-PS Converter2/1
  G2/1 -> Simulink-PS Converter1/1
  G1/1 -> Simulink-PS Converter/1
  connections:
  Simulink-PS Converter3/RConn1 -- MOSFETB2/LConn1
  Simulink-PS Converter2/RConn1 -- MOSFETB1/LConn1
  Simulink-PS Converter1/RConn1 -- MOSFETA2/LConn1
  Simulink-PS Converter/RConn1 -- MOSFETA1/LConn1
  MOSFETA2/RConn2 -- MOSFETB2/RConn2 -- N1/RConn1
  MOSFETA1/RConn1 -- MOSFETB1/RConn1 -- P1/RConn1
  MOSFETA1/RConn2 -- MOSFETA2/RConn1 -- P2/RConn1
  MOSFETB1/RConn2 -- MOSFETB2/RConn1 -- N2/RConn1

== system CLLCTestHarnessPlant/CLLC Converter Power Circuit/CLLCConverterVariant/SimplifiedModel/Secondary Converter/Subsystem4 ==
  PS-Simulink Converter : nesl_utility/PS-Simulink Converter  PhysicalDomain=network_engine_domain  SubClassName=ps_output  LeftPortType=input  RightPortType=output  PseudoPeriodic=off  Frequencies=[]  VectorFormat=inherit  Unit=inherit  AffineConversion=off
  Voltage Sensor : fl_lib/Electrical/Electrical Sensors/Voltage Sensor
  + : PMIOPort  Side=Left
  - : PMIOPort  Port=2  Side=Right
  V : Outport
  wires:
  PS-Simulink Converter/1 -> V/1
  connections:
  PS-Simulink Converter/LConn1 -- Voltage Sensor/RConn1
  Voltage Sensor/LConn1 -- +/RConn1
  Voltage Sensor/RConn2 -- -/RConn1

== system CLLCTestHarnessPlant/CLLC Converter Power Circuit/CLLCConverterVariant/SimplifiedModel/Secondary Converter/Vout ==
  PS-Simulink Converter : nesl_utility/PS-Simulink Converter  PhysicalDomain=network_engine_domain  SubClassName=ps_output  LeftPortType=input  RightPortType=output  PseudoPeriodic=off  Frequencies=[]  VectorFormat=inherit  Unit=inherit  AffineConversion=off
  Voltage Sensor : fl_lib/Electrical/Electrical Sensors/Voltage Sensor
  + : PMIOPort  Side=Left
  - : PMIOPort  Port=2  Side=Right
  V : Outport
  wires:
  PS-Simulink Converter/1 -> V/1
  connections:
  PS-Simulink Converter/LConn1 -- Voltage Sensor/RConn1
  Voltage Sensor/LConn1 -- +/RConn1
  Voltage Sensor/RConn2 -- -/RConn1

== system CLLCTestHarnessPlant/CLLC PWM Generator/Synchronous Rectifier/Turn On Delay/Rectifier Ramp Mode/FixedStep ==
  rate : Inport
  Rectifier Delay Timer : DiscreteIntegrator  SampleTime=Ts  LimitOutput=on  UpperSaturationLimit=Tsr  LowerSaturationLimit=0  ICPrevOutput=DiscIntNeverNeededParam  ICPrevScaledInput=DiscIntNeverNeededParam
  S : Outport
  wires:
  Rectifier Delay Timer/1 -> S/1
  rate/1 -> Rectifier Delay Timer/1

== system CLLCTestHarnessPlant/CLLC PWM Generator/Synchronous Rectifier/Turn On Delay/Rectifier Ramp Mode/VariableStep ==
  rate : Inport
  Rectifier Delay Timer : Integrator  LimitOutput=on  UpperSaturationLimit=Tsr  LowerSaturationLimit=0
  S : Outport
  wires:
  Rectifier Delay Timer/1 -> S/1
  rate/1 -> Rectifier Delay Timer/1
